simulink model "landing_gear_test"  (R2026b)
settings: Solver=ode4  StopTime=5  FixedStep=timestep
undefined symbols (not defined in the file): timestep
libraries: aerolibanimutils x1
settings Model: Creator=Teama  LastModifiedBy=Teama

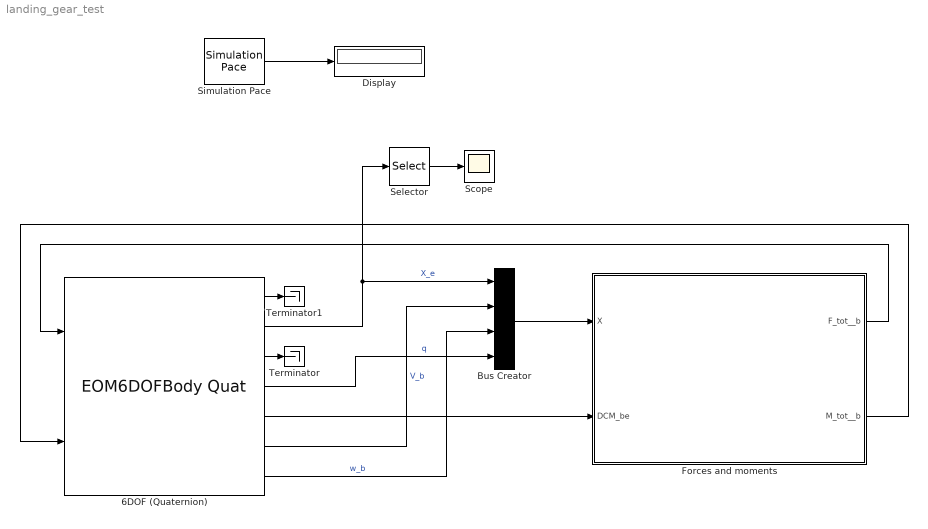
== system landing_gear_test ==
  6DOF (Quaternion) : EOM6DOFBodyQuat  xme_0=[0 0 -225]
  Bus Creator : BusCreator  Inputs=4
  Display : Display
  Forces and moments : Subsystem
  Scope : Scope
      settings: ActiveDisplayYMinimum=-225.17949901777948  ActiveDisplayYMaximum=-223.38450883998479
  Selector : Selector  InputPortWidth=3  IndexOptions=Index vector (dialog)  Indices=[3]  OutputSizes=1
  Simulation Pace : aerolibanimutils/Simulation Pace  SimulationPace=1  SleepMode=Auto  OutputPaceError=on  SampleTime=timestep
  Terminator : Terminator
  Terminator1 : Terminator
  wires:
  6DOF (Quaternion)/2 -> Selector/1, Bus Creator/1  "X_e"
  6DOF (Quaternion)/4 -> Bus Creator/4  "q"
  6DOF (Quaternion)/6 -> Bus Creator/2  "V_b"
  6DOF (Quaternion)/7 -> Bus Creator/3  "w_b"
  6DOF (Quaternion)/3 -> Terminator/1
  6DOF (Quaternion)/1 -> Terminator1/1
  Bus Creator/1 -> Forces and moments/1(X)
  6DOF (Quaternion)/5 -> Forces and moments/2(DCM_be)
  Forces and moments/1(F_tot__b) -> 6DOF (Quaternion)/1
  Forces and moments/2(M_tot__b) -> 6DOF (Quaternion)/2
  Selector/1 -> Scope/1
  Simulation Pace/1 -> Display/1

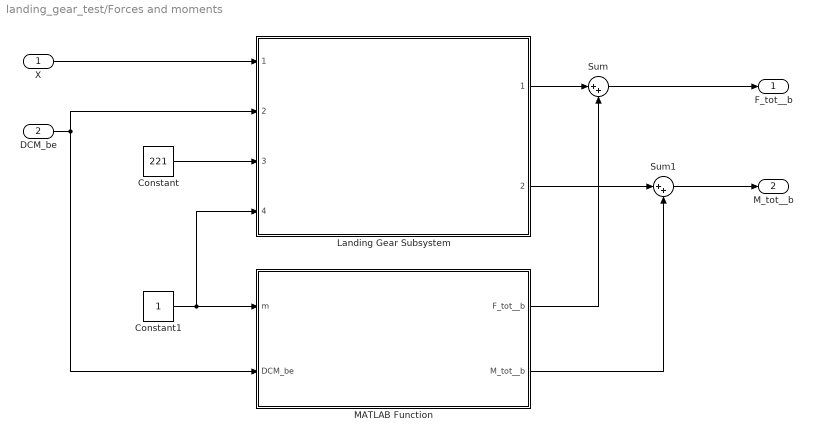
== system landing_gear_test/Forces and moments ==
  X : Inport
  DCM_be : Inport  Port=2
  Constant : Constant  Value=221
  Constant1 : Constant
  Landing Gear Subsystem : Subsystem  ReferencedSubsystem=Landing_Gear_Subsystem
  MATLAB Function : MATLAB Function  TreatAsAtomicUnit=on
  Sum : Sum  Inputs=|++
  Sum1 : Sum  Inputs=|++
  F_tot__b : Outport  OutDataTypeStr=double  PortDimensions=[3,1]
  M_tot__b : Outport  Port=2  OutDataTypeStr=double  PortDimensions=[3,1]
  wires:
  Constant/1 -> Landing Gear Subsystem/3
  DCM_be/1 -> MATLAB Function/2(DCM_be), Landing Gear Subsystem/2
  X/1 -> Landing Gear Subsystem/1
  Landing Gear Subsystem/2 -> Sum1/1
  Landing Gear Subsystem/1 -> Sum/1
  Constant1/1 -> Landing Gear Subsystem/4, MATLAB Function/1(m)
  MATLAB Function/1(F_tot__b) -> Sum/2
  Sum/1 -> F_tot__b/1
  MATLAB Function/2(M_tot__b) -> Sum1/2
  Sum1/1 -> M_tot__b/1

== matlab function landing_gear_test/Forces and moments/MATLAB Function ==
  data: m input; F_tot__b output double size=[3,1]; M_tot__b output double size=[3,1]; DCM_be input
function [F_tot__b, M_tot__b] = gravity_wrapper(m, DCM_be)
    F_tot__b = zeros(3,1);
    M_tot__b = zeros(3,1);

    [F_tot__b, M_tot__b] = gravity(m, DCM_be);
end
